simulink model "afe_rst_inv_psm_distributed_control_two_delays"  (R2026a)
settings: Solver=ode1be  StopTime=simlength  FixedStep=tc  MaxStep=Tc
values from neighbouring files (symbols this model uses):
  Amplitude_U = 1.16    [grid_fault_generator.m]
  Amplitude_V = Amplitude_U    (= 1.16)    [grid_fault_generator.m]
  Amplitude_W = Amplitude_U    (= 1.16)    [grid_fault_generator.m]
  end_time_LVRT = start_time_LVRT + error_length    [grid_fault_generator.m]
  Igrid_phase_normalization_factor = 270*sqrt(2)    [grid_emulator.m]
  omega_grid_emulator_nom = w_grid    (= 314.159265359)    [grid_emulator.m]
  omega_grid_nom = w_grid    (= 314.159265359)    [grid_emulator.m]
  t_ramp = 20e-3    (= 0.02)    [grid_fault_generator.m]
  ugrid_factor = 1    [grid_emulator.m]
  V_phase_normalization_factor = Vgrid_phase_normalization_factor    [grid_emulator.m]
  Vdc_bez = 1070    [grid_emulator.m]
  Vemu_ref_norm = Vemu_ref * sqrt(2) / V_phase_normalization_factor    [grid_emulator.m]
  vn_eta_pu = 0    [grid_emulator.m]
  vn_xi_pu = 0    [grid_emulator.m]
  vp_xi_pu = 1    [grid_emulator.m]
undefined symbols (not defined in the file or in its folder): Adrso, Aresd, Bresd, CFi, CFu, Cresd, Crso, CTRPIFF_CLIP_RELEASE, dead_time_INV, emf_fb_p, emf_fb_p_ccaller_1, emf_fb_p_ccaller_2, emf_p, emf_p_ccaller_1, emf_p_ccaller_2, fPWM_INV, g0_161Hz, g0_500Hz, g1_161Hz, g1_500Hz, i_grid_neg_eta_lim, i_grid_neg_eta_red_lim, i_grid_neg_xi_lim, i_grid_neg_xi_red_lim, i_grid_pos_eta_lim, i_grid_pos_eta_red_lim, ibez, id_lim, ieta_neg_ref_lim, ieta_pos_ref_lim, iq_lim, ixi_pos_ref_lim, Jm_norm, k_frt_ref, kg, ki_afe, ki_i, ki_id, ki_iq, ki_rc_neg_grid, ki_rc_pos_grid, ki_vs, ki_w, kp_afe, kp_i, kp_id, kp_iq, kp_rc_neg_grid, kp_rc_pos_grid, kp_vs, kp_w, kw, l1, l2, Lalpha_norm, Ld_norm, Ldrso, Lq_norm, Ls_norm, luenberger_l1 ... (+30)
libraries: fl_lib x146, nesl_utility x62, simulink x8, cstblocks_lti x7, sl_discontinuities x3, single_phase_transformer_lib x3, flexshaft_lib x1, permanent_magnet_synchronous_machine x1
(part 5 of 14)

== system afe_rst_inv_psm_distributed_control_two_delays/mainboard_afe/sequences_current_control/negative_sequence_xi_current_control ==
  ff : Inport
  e : Inport  Port=2
  1/Ti : Gain  Gain=kp_rc_neg_grid  SaturateOnIntegerOverflow=on  OutDataTypeStr=Inherit: Same as input  ParamDataTypeStr=Inherit: Same as input
  1/Ti1 : Gain  SaturateOnIntegerOverflow=on  OutDataTypeStr=Inherit: Same as input  ParamDataTypeStr=Inherit: Same as input
  Saturation : Saturate  UpperLimit=ieta_pos_ref_lim  LowerLimit=-ieta_pos_ref_lim
  Sum : Sum  Inputs=|++
  Sum2 : Sum  Inputs=+++  SaturateOnIntegerOverflow=on
  Sum3 : Sum  Inputs=-+  SaturateOnIntegerOverflow=on
  Unit Delay1 : UnitDelay  SampleTime=ts_afe
  Unit Delay4 : UnitDelay  SampleTime=ts_afe
  kp : Gain  Gain=ki_rc_neg_grid*ts_afe  SaturateOnIntegerOverflow=on  OutDataTypeStr=Inherit: Same as input  ParamDataTypeStr=Inherit: Same as input
  u : Outport  VectorParamsAs1DForOutWhenUnconnected=off
  wires:
  Unit Delay4/1 -> Sum2/3
  Sum3/1 -> Unit Delay4/1
  kp/1 -> Sum2/2
  Sum2/1 -> Saturation/1
  1/Ti/1 -> Sum2/1, Sum3/1
  Saturation/1 -> Sum/1, Sum3/2
  Sum/1 -> Unit Delay1/1
  ff/1 -> 1/Ti1/1
  1/Ti1/1 -> Sum/2
  e/1 -> 1/Ti/1, kp/1  "e"
  Unit Delay1/1 -> u/1

== system afe_rst_inv_psm_distributed_control_two_delays/mainboard_afe/sequences_current_control/positive_sequence_eta_current_control ==
  ff : Inport
  e : Inport  Port=2
  1/Ti : Gain  Gain=kp_rc_pos_grid  SaturateOnIntegerOverflow=on  OutDataTypeStr=Inherit: Same as input  ParamDataTypeStr=Inherit: Same as input
  1/Ti1 : Gain  SaturateOnIntegerOverflow=on  OutDataTypeStr=Inherit: Same as input  ParamDataTypeStr=Inherit: Same as input
  Saturation : Saturate  UpperLimit=ieta_pos_ref_lim  LowerLimit=-ieta_pos_ref_lim
  Sum : Sum  Inputs=|++
  Sum2 : Sum  Inputs=+++  SaturateOnIntegerOverflow=on
  Sum3 : Sum  Inputs=-+  SaturateOnIntegerOverflow=on
  Unit Delay1 : UnitDelay  SampleTime=ts_afe
  Unit Delay4 : UnitDelay  SampleTime=ts_afe
  kp : Gain  Gain=ki_rc_pos_grid*ts_afe  SaturateOnIntegerOverflow=on  OutDataTypeStr=Inherit: Same as input  ParamDataTypeStr=Inherit: Same as input
  u : Outport  VectorParamsAs1DForOutWhenUnconnected=off
  wires:
  Unit Delay4/1 -> Sum2/3
  Sum3/1 -> Unit Delay4/1
  kp/1 -> Sum2/2
  Sum2/1 -> Saturation/1
  1/Ti/1 -> Sum2/1, Sum3/1
  Saturation/1 -> Sum/1, Sum3/2
  ff/1 -> 1/Ti1/1
  1/Ti1/1 -> Sum/2
  e/1 -> 1/Ti/1, kp/1  "e"
  Sum/1 -> Unit Delay1/1
  Unit Delay1/1 -> u/1

== system afe_rst_inv_psm_distributed_control_two_delays/mainboard_afe/voltage-current-acquisition/iga_fieldbus ==
  is : Inport
  Unit Delay : UnitDelay  SampleTime=ts_afe
  Unit Delay1 : UnitDelay  SampleTime=ts_afe
  Zero-Order Hold : ZeroOrderHold  SampleTime=ts_afe
  is_fb : Outport
  wires:
  is/1 -> Zero-Order Hold/1
  Unit Delay/1 -> Unit Delay1/1
  Zero-Order Hold/1 -> Unit Delay/1
  Unit Delay1/1 -> is_fb/1

== system afe_rst_inv_psm_distributed_control_two_delays/mainboard_afe/voltage-current-acquisition/igb_fieldbus ==
  is : Inport
  Unit Delay : UnitDelay  SampleTime=ts_afe
  Unit Delay1 : UnitDelay  SampleTime=ts_afe
  Zero-Order Hold : ZeroOrderHold  SampleTime=ts_afe
  is_fb : Outport
  wires:
  is/1 -> Zero-Order Hold/1
  Unit Delay/1 -> Unit Delay1/1
  Zero-Order Hold/1 -> Unit Delay/1
  Unit Delay1/1 -> is_fb/1

== system afe_rst_inv_psm_distributed_control_two_delays/mainboard_afe/voltage-current-acquisition/igc_fieldbus ==
  is : Inport
  Unit Delay : UnitDelay  SampleTime=ts_afe
  Unit Delay1 : UnitDelay  SampleTime=ts_afe
  Zero-Order Hold : ZeroOrderHold  SampleTime=ts_afe
  is_fb : Outport
  wires:
  is/1 -> Zero-Order Hold/1
  Unit Delay/1 -> Unit Delay1/1
  Zero-Order Hold/1 -> Unit Delay/1
  Unit Delay1/1 -> is_fb/1

== system afe_rst_inv_psm_distributed_control_two_delays/mainboard_afe/voltage-current-acquisition/isa_fieldbus ==
  is : Inport
  Unit Delay : UnitDelay  SampleTime=ts_afe
  Unit Delay1 : UnitDelay  SampleTime=ts_afe
  Zero-Order Hold : ZeroOrderHold  SampleTime=ts_afe
  is_fb : Outport
  wires:
  is/1 -> Zero-Order Hold/1
  Unit Delay/1 -> Unit Delay1/1
  Zero-Order Hold/1 -> Unit Delay/1
  Unit Delay1/1 -> is_fb/1

== system afe_rst_inv_psm_distributed_control_two_delays/mainboard_afe/voltage-current-acquisition/isb_fieldbus ==
  is : Inport
  Unit Delay : UnitDelay  SampleTime=ts_afe
  Unit Delay1 : UnitDelay  SampleTime=ts_afe
  Zero-Order Hold : ZeroOrderHold  SampleTime=ts_afe
  is_fb : Outport
  wires:
  is/1 -> Zero-Order Hold/1
  Unit Delay/1 -> Unit Delay1/1
  Zero-Order Hold/1 -> Unit Delay/1
  Unit Delay1/1 -> is_fb/1

== system afe_rst_inv_psm_distributed_control_two_delays/mainboard_afe/voltage-current-acquisition/isc_fieldbus ==
  is : Inport
  Unit Delay : UnitDelay  SampleTime=ts_afe
  Unit Delay1 : UnitDelay  SampleTime=ts_afe
  Zero-Order Hold : ZeroOrderHold  SampleTime=ts_afe
  is_fb : Outport
  wires:
  is/1 -> Zero-Order Hold/1
  Unit Delay/1 -> Unit Delay1/1
  Zero-Order Hold/1 -> Unit Delay/1
  Unit Delay1/1 -> is_fb/1

== system afe_rst_inv_psm_distributed_control_two_delays/mainboard_afe/voltage-current-acquisition/uga_fieldbus ==
  ug : Inport
  Unit Delay : UnitDelay  SampleTime=ts_afe
  Unit Delay1 : UnitDelay  SampleTime=ts_afe
  Zero-Order Hold : ZeroOrderHold  SampleTime=ts_afe
  ug_fb : Outport
  wires:
  ug/1 -> Zero-Order Hold/1
  Unit Delay/1 -> Unit Delay1/1
  Zero-Order Hold/1 -> Unit Delay/1
  Unit Delay1/1 -> ug_fb/1

== system afe_rst_inv_psm_distributed_control_two_delays/mainboard_afe/voltage-current-acquisition/ugb_fieldbus ==
  ug : Inport
  Unit Delay : UnitDelay  SampleTime=ts_afe
  Unit Delay1 : UnitDelay  SampleTime=ts_afe
  Zero-Order Hold : ZeroOrderHold  SampleTime=ts_afe
  ug_fb : Outport
  wires:
  ug/1 -> Zero-Order Hold/1
  Unit Delay/1 -> Unit Delay1/1
  Zero-Order Hold/1 -> Unit Delay/1
  Unit Delay1/1 -> ug_fb/1

== system afe_rst_inv_psm_distributed_control_two_delays/mainboard_afe/voltage-current-acquisition/ugb_fieldbus1 ==
  ug : Inport
  Unit Delay : UnitDelay  SampleTime=ts_afe
  Unit Delay1 : UnitDelay  SampleTime=ts_afe
  Zero-Order Hold : ZeroOrderHold  SampleTime=ts_afe
  ug_fb : Outport
  wires:
  ug/1 -> Zero-Order Hold/1
  Unit Delay/1 -> Unit Delay1/1
  Zero-Order Hold/1 -> Unit Delay/1
  Unit Delay1/1 -> ug_fb/1

== system afe_rst_inv_psm_distributed_control_two_delays/mainboard_afe/voltage_sequence_avg/Moving Average Filter1 ==
  In2 : Inport
  In3 : Inport  Port=2
  Bus Selector : BusSelector  OutputSignals=ts,sshort,slong,pinput,cbpointer,cbsample,mavg_output
  C Caller : CCaller  FunctionName=mavgflt_process_simulink  PortSpecificationStruct="%)30     .    B H   8    (     @         %    \"     8    !     0         %  0 \"0    $    _    07)G3F%M90  4&]R=$YA;64 4V-O<&4     26YD97@     5'EP90      4VEZ90      27-';&]B86P   X    P    !@    @    $          4    (     0    ,    !         !   P!O=70 #@   #     &    \"     0         !0    @    !     P    $         $  # &]U=  .    .     8    (    !          %    \"     $    &     0         0   ...(+3251 chars)"  SampleTime=ts_afe
  Compare To Zero : simulink/Logic and Bit Operations/Compare To Zero  relop=>  OutDataTypeStr=boolean
  Constant : Constant
  Constant5 : Constant  Value=ts_afe
  Data Type Conversion : DataTypeConversion  OutDataTypeStr=single  SaturateOnIntegerOverflow=off  RndMeth=Floor
  Data Type Conversion1 : DataTypeConversion  OutDataTypeStr=single  SaturateOnIntegerOverflow=off  RndMeth=Floor
  Data Type Conversion2 : DataTypeConversion  OutDataTypeStr=single  SaturateOnIntegerOverflow=off  RndMeth=Floor
  Data Type Conversion3 : DataTypeConversion  OutDataTypeStr=double  SaturateOnIntegerOverflow=off  RndMeth=Floor
  Data Type Conversion4 : DataTypeConversion  OutDataTypeStr=uint8  SaturateOnIntegerOverflow=off  RndMeth=Floor
  Data Type Conversion5 : DataTypeConversion  OutDataTypeStr=uint8  SaturateOnIntegerOverflow=off  RndMeth=Floor
  Enabled Subsystem : Subsystem  TreatAsAtomicUnit=on
  Reset Trigger : Subsystem
  Terminator{,1..5} (6 alike) : Terminator
  Zero-Order Hold1 : ZeroOrderHold  SampleTime=ts_afe
  Zero-Order Hold2 : ZeroOrderHold  SampleTime=ts_afe
  xi : Outport
  wires:
  Bus Selector/5 -> Terminator2/1  "<cbpointer>"
  Bus Selector/4 -> Terminator1/1  "<pinput>"
  Data Type Conversion3/1 -> xi/1  "output"
  Zero-Order Hold2/1 -> Data Type Conversion/1  "d1"
  Enabled Subsystem/1(Out1) -> Data Type Conversion1/1
  Compare To Zero/1 -> Enabled Subsystem/Enable
  In3/1 -> Enabled Subsystem/1(In1), Compare To Zero/1  "omega_grid"
  Constant5/1 -> Zero-Order Hold1/1
  Zero-Order Hold1/1 -> Data Type Conversion2/1  "d1"
  Bus Selector/3 -> Terminator4/1  "<slong>"
  Bus Selector/2 -> Terminator3/1  "<sshort>"
  Bus Selector/1 -> Terminator/1  "<ts>"
  C Caller/1 -> Bus Selector/1  "out"
  In2/1 -> Zero-Order Hold2/1  "input"
  Data Type Conversion4/1 -> C Caller/5
  Data Type Conversion/1 -> C Caller/1  "input"
  Data Type Conversion5/1 -> C Caller/4
  Data Type Conversion2/1 -> C Caller/3
  Data Type Conversion1/1 -> C Caller/2
  Reset Trigger/1(Out1) -> Data Type Conversion5/1
  Constant/1 -> Data Type Conversion4/1
  Bus Selector/6 -> Terminator5/1  "<cbsample>"
  Bus Selector/7 -> Data Type Conversion3/1  "<mavg_output>"

== system afe_rst_inv_psm_distributed_control_two_delays/mainboard_afe/voltage_sequence_avg/Moving Average Filter2 ==
  In2 : Inport
  In3 : Inport  Port=2
  Bus Selector : BusSelector  OutputSignals=ts,sshort,slong,pinput,cbpointer,cbsample,mavg_output
  C Caller : CCaller  FunctionName=mavgflt_process_simulink  PortSpecificationStruct="%)30     .    B H   8    (     @         %    \"     8    !     0         %  0 \"0    $    _    07)G3F%M90  4&]R=$YA;64 4V-O<&4     26YD97@     5'EP90      4VEZ90      27-';&]B86P   X    P    !@    @    $          4    (     0    ,    !         !   P!O=70 #@   #     &    \"     0         !0    @    !     P    $         $  # &]U=  .    .     8    (    !          %    \"     $    &     0         0   ...(+3251 chars)"  SampleTime=ts_afe
  Compare To Zero : simulink/Logic and Bit Operations/Compare To Zero  relop=>  OutDataTypeStr=boolean
  Constant : Constant  Value=2
  Constant5 : Constant  Value=ts_afe
  Data Type Conversion : DataTypeConversion  OutDataTypeStr=single  SaturateOnIntegerOverflow=off  RndMeth=Floor
  Data Type Conversion1 : DataTypeConversion  OutDataTypeStr=single  SaturateOnIntegerOverflow=off  RndMeth=Floor
  Data Type Conversion2 : DataTypeConversion  OutDataTypeStr=single  SaturateOnIntegerOverflow=off  RndMeth=Floor
  Data Type Conversion3 : DataTypeConversion  OutDataTypeStr=double  SaturateOnIntegerOverflow=off  RndMeth=Floor
  Data Type Conversion4 : DataTypeConversion  OutDataTypeStr=uint8  SaturateOnIntegerOverflow=off  RndMeth=Floor
  Data Type Conversion5 : DataTypeConversion  OutDataTypeStr=uint8  SaturateOnIntegerOverflow=off  RndMeth=Floor
  Enabled Subsystem : Subsystem  TreatAsAtomicUnit=on
  Reset Trigger : Subsystem
  Terminator{,1..5} (6 alike) : Terminator
  Zero-Order Hold1 : ZeroOrderHold  SampleTime=ts_afe
  Zero-Order Hold2 : ZeroOrderHold  SampleTime=ts_afe
  xi : Outport
  wires:
  Bus Selector/7 -> Data Type Conversion3/1  "<mavg_output>"
  Bus Selector/6 -> Terminator5/1  "<cbsample>"
  Constant/1 -> Data Type Conversion4/1
  Reset Trigger/1(Out1) -> Data Type Conversion5/1
  Data Type Conversion1/1 -> C Caller/2
  Data Type Conversion2/1 -> C Caller/3
  Data Type Conversion5/1 -> C Caller/4
  Data Type Conversion/1 -> C Caller/1  "input"
  Data Type Conversion4/1 -> C Caller/5
  In2/1 -> Zero-Order Hold2/1  "input"
  C Caller/1 -> Bus Selector/1  "out"
  Bus Selector/1 -> Terminator/1  "<ts>"
  Bus Selector/2 -> Terminator3/1  "<sshort>"
  Bus Selector/3 -> Terminator4/1  "<slong>"
  Zero-Order Hold1/1 -> Data Type Conversion2/1  "d1"
  Constant5/1 -> Zero-Order Hold1/1
  In3/1 -> Compare To Zero/1, Enabled Subsystem/1(In1)  "omega_grid"
  Compare To Zero/1 -> Enabled Subsystem/Enable
  Enabled Subsystem/1(Out1) -> Data Type Conversion1/1
  Zero-Order Hold2/1 -> Data Type Conversion/1  "d1"
  Data Type Conversion3/1 -> xi/1  "output"
  Bus Selector/4 -> Terminator1/1  "<pinput>"
  Bus Selector/5 -> Terminator2/1  "<cbpointer>"

== system afe_rst_inv_psm_distributed_control_two_delays/mainboard_afe/voltage_sequence_avg/Moving Average Filter3 ==
  In2 : Inport
  In3 : Inport  Port=2
  Bus Selector : BusSelector  OutputSignals=ts,sshort,slong,pinput,cbpointer,cbsample,mavg_output
  C Caller : CCaller  FunctionName=mavgflt_process_simulink  PortSpecificationStruct="%)30     .    B H   8    (     @         %    \"     8    !     0         %  0 \"0    $    _    07)G3F%M90  4&]R=$YA;64 4V-O<&4     26YD97@     5'EP90      4VEZ90      27-';&]B86P   X    P    !@    @    $          4    (     0    ,    !         !   P!O=70 #@   #     &    \"     0         !0    @    !     P    $         $  # &]U=  .    .     8    (    !          %    \"     $    &     0         0   ...(+3251 chars)"  SampleTime=ts_afe
  Compare To Zero : simulink/Logic and Bit Operations/Compare To Zero  relop=>  OutDataTypeStr=boolean
  Constant : Constant  Value=3
  Constant5 : Constant  Value=ts_afe
  Data Type Conversion : DataTypeConversion  OutDataTypeStr=single  SaturateOnIntegerOverflow=off  RndMeth=Floor
  Data Type Conversion1 : DataTypeConversion  OutDataTypeStr=single  SaturateOnIntegerOverflow=off  RndMeth=Floor
  Data Type Conversion2 : DataTypeConversion  OutDataTypeStr=single  SaturateOnIntegerOverflow=off  RndMeth=Floor
  Data Type Conversion3 : DataTypeConversion  OutDataTypeStr=double  SaturateOnIntegerOverflow=off  RndMeth=Floor
  Data Type Conversion4 : DataTypeConversion  OutDataTypeStr=uint8  SaturateOnIntegerOverflow=off  RndMeth=Floor
  Data Type Conversion5 : DataTypeConversion  OutDataTypeStr=uint8  SaturateOnIntegerOverflow=off  RndMeth=Floor
  Enabled Subsystem : Subsystem  TreatAsAtomicUnit=on
  Reset Trigger : Subsystem
  Terminator{,1..5} (6 alike) : Terminator
  Zero-Order Hold1 : ZeroOrderHold  SampleTime=ts_afe
  Zero-Order Hold2 : ZeroOrderHold  SampleTime=ts_afe
  xi : Outport
  wires:
  Bus Selector/5 -> Terminator2/1  "<cbpointer>"
  Bus Selector/4 -> Terminator1/1  "<pinput>"
  Data Type Conversion3/1 -> xi/1  "output"
  Zero-Order Hold2/1 -> Data Type Conversion/1  "d1"
  Enabled Subsystem/1(Out1) -> Data Type Conversion1/1
  Compare To Zero/1 -> Enabled Subsystem/Enable
  In3/1 -> Enabled Subsystem/1(In1), Compare To Zero/1  "omega_grid"
  Constant5/1 -> Zero-Order Hold1/1
  Zero-Order Hold1/1 -> Data Type Conversion2/1  "d1"
  Bus Selector/3 -> Terminator4/1  "<slong>"
  Bus Selector/2 -> Terminator3/1  "<sshort>"
  Bus Selector/1 -> Terminator/1  "<ts>"
  C Caller/1 -> Bus Selector/1  "out"
  In2/1 -> Zero-Order Hold2/1  "input"
  Data Type Conversion4/1 -> C Caller/5
  Data Type Conversion/1 -> C Caller/1  "input"
  Data Type Conversion5/1 -> C Caller/4
  Data Type Conversion2/1 -> C Caller/3
  Data Type Conversion1/1 -> C Caller/2
  Reset Trigger/1(Out1) -> Data Type Conversion5/1
  Constant/1 -> Data Type Conversion4/1
  Bus Selector/6 -> Terminator5/1  "<cbsample>"
  Bus Selector/7 -> Data Type Conversion3/1  "<mavg_output>"

== system afe_rst_inv_psm_distributed_control_two_delays/mainboard_afe/voltage_sequence_avg/Moving Average Filter4 ==
  In2 : Inport
  In3 : Inport  Port=2
  Bus Selector : BusSelector  OutputSignals=ts,sshort,slong,pinput,cbpointer,cbsample,mavg_output
  C Caller : CCaller  FunctionName=mavgflt_process_simulink  PortSpecificationStruct="%)30     .    B H   8    (     @         %    \"     8    !     0         %  0 \"0    $    _    07)G3F%M90  4&]R=$YA;64 4V-O<&4     26YD97@     5'EP90      4VEZ90      27-';&]B86P   X    P    !@    @    $          4    (     0    ,    !         !   P!O=70 #@   #     &    \"     0         !0    @    !     P    $         $  # &]U=  .    .     8    (    !          %    \"     $    &     0         0   ...(+3251 chars)"  SampleTime=ts_afe
  Compare To Zero : simulink/Logic and Bit Operations/Compare To Zero  relop=>  OutDataTypeStr=boolean
  Constant : Constant  Value=4
  Constant5 : Constant  Value=ts_afe
  Data Type Conversion : DataTypeConversion  OutDataTypeStr=single  SaturateOnIntegerOverflow=off  RndMeth=Floor
  Data Type Conversion1 : DataTypeConversion  OutDataTypeStr=single  SaturateOnIntegerOverflow=off  RndMeth=Floor
  Data Type Conversion2 : DataTypeConversion  OutDataTypeStr=single  SaturateOnIntegerOverflow=off  RndMeth=Floor
  Data Type Conversion3 : DataTypeConversion  OutDataTypeStr=double  SaturateOnIntegerOverflow=off  RndMeth=Floor
  Data Type Conversion4 : DataTypeConversion  OutDataTypeStr=uint8  SaturateOnIntegerOverflow=off  RndMeth=Floor
  Data Type Conversion5 : DataTypeConversion  OutDataTypeStr=uint8  SaturateOnIntegerOverflow=off  RndMeth=Floor
  Enabled Subsystem : Subsystem  TreatAsAtomicUnit=on
  Reset Trigger : Subsystem
  Terminator{,1..5} (6 alike) : Terminator
  Zero-Order Hold1 : ZeroOrderHold  SampleTime=ts_afe
  Zero-Order Hold2 : ZeroOrderHold  SampleTime=ts_afe
  xi : Outport
  wires:
  Bus Selector/7 -> Data Type Conversion3/1  "<mavg_output>"
  Bus Selector/6 -> Terminator5/1  "<cbsample>"
  Constant/1 -> Data Type Conversion4/1
  Reset Trigger/1(Out1) -> Data Type Conversion5/1
  Data Type Conversion1/1 -> C Caller/2
  Data Type Conversion2/1 -> C Caller/3
  Data Type Conversion5/1 -> C Caller/4
  Data Type Conversion/1 -> C Caller/1  "input"
  Data Type Conversion4/1 -> C Caller/5
  In2/1 -> Zero-Order Hold2/1  "input"
  C Caller/1 -> Bus Selector/1  "out"
  Bus Selector/1 -> Terminator/1  "<ts>"
  Bus Selector/2 -> Terminator3/1  "<sshort>"
  Bus Selector/3 -> Terminator4/1  "<slong>"
  Zero-Order Hold1/1 -> Data Type Conversion2/1  "d1"
  Constant5/1 -> Zero-Order Hold1/1
  In3/1 -> Compare To Zero/1, Enabled Subsystem/1(In1)  "omega_grid"
  Compare To Zero/1 -> Enabled Subsystem/Enable
  Enabled Subsystem/1(Out1) -> Data Type Conversion1/1
  Zero-Order Hold2/1 -> Data Type Conversion/1  "d1"
  Data Type Conversion3/1 -> xi/1  "output"
  Bus Selector/4 -> Terminator1/1  "<pinput>"
  Bus Selector/5 -> Terminator2/1  "<cbpointer>"

== system afe_rst_inv_psm_distributed_control_two_delays/AFE-Modular/afe_leg_a/driver_board_a/current_ctrl ==
  i_xi_ref : Inport
  phase_current_control : Subsystem
  xieta2abc : Subsystem
  us_alphabeta_ctrl : Outport
  wires:
  i_xi_ref/1 -> xieta2abc/1(pos_xi)  "i_xi_ref"
  phase_current_control/1(us_alphabeta_ctrl) -> us_alphabeta_ctrl/1
  xieta2abc/1(i_abc) -> phase_current_control/1(In1)  "is_abc_reference"
  [gamma_grid_phase_a] -> xieta2abc/5(gamma)
  [isa_pu_dba] -> phase_current_control/2(is_abc)
  [is_eta_pos_ref_mb_fb_dba] -> xieta2abc/2(pos_eta)
  [is_xi_neg_ref_mb_fb_dba] -> xieta2abc/3(neg_xi)
  [is_eta_neg_ref_mb_fb_dba] -> xieta2abc/4(neg_eta)

== system afe_rst_inv_psm_distributed_control_two_delays/AFE-Modular/afe_leg_a/driver_board_a/dq_pll ==
  pll_stageA : Subsystem
  pll_stageB : Subsystem
  tag scope: gamma_grid_phase_a=global
  wires:
  pll_stageB/1(gamma_grid_pll) -> pll_stageA/1(gamma_grid), [gamma_grid_phase_a]
  pll_stageA/2(u_grid_pos_eta) -> pll_stageB/2(u_grid_pos_eta)  "u_grid_pos_eta"
  pll_stageA/1(u_grid_pos_xi) -> pll_stageB/1(u_grid_pos_xi)  "u_grid_pos_xi"

== system afe_rst_inv_psm_distributed_control_two_delays/AFE-Modular/afe_leg_a/driver_board_a/iga_dba_estimator ==
  Gain : Gain  Gain=omega_grid_nom*CFu
  Sum : Sum  Inputs=|++
  quadrature_shift_filter : MATLAB Function  TreatAsAtomicUnit=on  SystemSampleTime=ts_afe
  tag scope: iga_pu_dba=global
  wires:
  Sum/1 -> [iga_pu_dba]
  quadrature_shift_filter/1(y) -> Sum/2
  [uga_pu_dba] -> Gain/1
  [isa_pu_dba] -> Sum/1
  Gain/1 -> quadrature_shift_filter/1(input)

== system afe_rst_inv_psm_distributed_control_two_delays/AFE-Modular/afe_leg_a/driver_board_a/udc_ctrl ==
  udc_pu : Inport
  udc_pu_ref : Inport  Port=2
  1/Ti : Gain  Gain=kp_vs  SaturateOnIntegerOverflow=on  OutDataTypeStr=Inherit: Same as input  ParamDataTypeStr=Inherit: Same as input
  Gain : Gain  Gain=-1
  Saturation : Saturate  UpperLimit=ixi_pos_ref_lim  LowerLimit=-ixi_pos_ref_lim
  Sum1 : Sum  Inputs=+++  SaturateOnIntegerOverflow=on
  Sum2 : Sum  Inputs=-+  SaturateOnIntegerOverflow=on
  Sum3 : Sum  Inputs=-+  SaturateOnIntegerOverflow=on
  Unit Delay4 : UnitDelay  SampleTime=ts_afe
  kp : Gain  Gain=ki_vs*ts_afe  SaturateOnIntegerOverflow=on  OutDataTypeStr=Inherit: Same as input  ParamDataTypeStr=Inherit: Same as input
  i_xi_ref : Outport
  wires:
  1/Ti/1 -> Sum1/1, Sum3/1
  kp/1 -> Sum1/2
  Sum3/1 -> Unit Delay4/1
  Unit Delay4/1 -> Sum1/3
  udc_pu_ref/1 -> Sum2/2
  udc_pu/1 -> Sum2/1
  Sum2/1 -> kp/1, 1/Ti/1
  Sum1/1 -> Saturation/1
  Saturation/1 -> Gain/1, Sum3/2
  Gain/1 -> i_xi_ref/1

== system afe_rst_inv_psm_distributed_control_two_delays/AFE-Modular/afe_leg_a/driver_board_a/voltage-current-acquisition ==
  is_eta_neg_ref_fieldbus : Subsystem
  is_eta_pos_ref_fieldbus : Subsystem
  is_xi_neg_ref_fieldbus : Subsystem
  isa_measure : Subsystem
  isb_fieldbus : Subsystem
  isc_fieldbus : Subsystem
  ixi_ref_fieldbus : Subsystem
  ixi_ref_fieldbus1 : Subsystem
  ub_ctrl_fieldbus : Subsystem
  uc_ctrl_fieldbus : Subsystem
  uga_measure : Subsystem
  ugb_fieldbus : Subsystem
  ugc_fieldbus : Subsystem
  tag scope: is_eta_neg_ref_mb_fb_dba=global, is_eta_pos_ref_mb_fb_dba=global, is_xi_neg_ref_mb_fb_dba=global, isa_pu_dba=global, isb_pu_dbb_fb_dba=global, isc_pu_dbc_fb_dba=global, ixi_ref_dbb_fb_dba=global, ixi_ref_dbc_fb_dba=global, uga_pu_dba=global, ugb_pu_dbb_fb_dba=global, ugc_pu_dbc_fb_dba=global, usb_ctrl_dbb_fb_dba=global, usc_ctrl_dbc_fb_dba=global
  wires:
  ub_ctrl_fieldbus/1(u_ctrl_fb) -> [usb_ctrl_dbb_fb_dba]
  [isc_pu_dbc] -> isc_fieldbus/1(is)
  isb_fieldbus/1(is_fb) -> [isb_pu_dbb_fb_dba]
  [usc_ctrl_dbc] -> uc_ctrl_fieldbus/1(u_ctrl)
  isa_measure/1(is_pu) -> [isa_pu_dba]
  [isb_pu_dbb] -> isb_fieldbus/1(is)
  [usb_ctrl_dbb] -> ub_ctrl_fieldbus/1(u_ctrl)
  [isa_dba] -> isa_measure/1(is)
  uc_ctrl_fieldbus/1(u_ctrl_fb) -> [usc_ctrl_dbc_fb_dba]
  isc_fieldbus/1(is_fb) -> [isc_pu_dbc_fb_dba]
  [uga_dba] -> uga_measure/1(ug)
  uga_measure/1(ug_pu) -> [uga_pu_dba]
  [ugc_pu_dbc] -> ugc_fieldbus/1(ug)
  [ugb_pu_dbb] -> ugb_fieldbus/1(ug)
  ugc_fieldbus/1(ug_fb) -> [ugc_pu_dbc_fb_dba]
  ugb_fieldbus/1(ug_fb) -> [ugb_pu_dbb_fb_dba]
  ixi_ref_fieldbus/1(is_fb) -> [ixi_ref_dbb_fb_dba]
  ixi_ref_fieldbus1/1(is_fb) -> [ixi_ref_dbc_fb_dba]
  [ixi_ref_dbc] -> ixi_ref_fieldbus1/1(is)
  [ixi_ref_dbb] -> ixi_ref_fieldbus/1(is)
  [i_stack_pos_eta_ref] -> is_eta_pos_ref_fieldbus/1(is)
  is_eta_pos_ref_fieldbus/1(is_fb) -> [is_eta_pos_ref_mb_fb_dba]
  [i_stack_neg_eta_ref] -> is_eta_neg_ref_fieldbus/1(is)
  is_eta_neg_ref_fieldbus/1(is_fb) -> [is_eta_neg_ref_mb_fb_dba]
  [i_stack_neg_xi_ref] -> is_xi_neg_ref_fieldbus/1(is)
  is_xi_neg_ref_fieldbus/1(is_fb) -> [is_xi_neg_ref_mb_fb_dba]

== system afe_rst_inv_psm_distributed_control_two_delays/AFE-Modular/afe_leg_a/modulator/sv_pwm ==
  ab : Inport
  enable : Inport  Port=2
  Bus Selector : BusSelector  OutputSignals=da,db,dc
  Bus Selector1 : BusSelector  OutputSignals=us_alpha_ctrl,us_beta_ctrl
  C Caller : CCaller  FunctionName=sv_pwm_process_simulink  PortSpecificationStruct="%)30     .    N @   8    (     @         %    \"     4    !     0         %  0 \"0    $    _    07)G3F%M90  4&]R=$YA;64 4V-O<&4     26YD97@     5'EP90      4VEZ90      27-';&]B86P   X    P    !@    @    $          4    (     0    ,    !         !   P!O=70 #@   #     &    \"     0         !0    @    !     P    $         $  # &]U=  .    .     8    (    !          %    \"     $    &     0         0   ...(+2630 chars)"  SampleTime=ts_afe
  Constant : Constant  Value=ts_afe
  Data Type Conversion1 : DataTypeConversion  OutDataTypeStr=double  SaturateOnIntegerOverflow=off  RndMeth=Floor
  Data Type Conversion15 : DataTypeConversion  OutDataTypeStr=single  SaturateOnIntegerOverflow=off  RndMeth=Floor
  Data Type Conversion16 : DataTypeConversion  OutDataTypeStr=single  SaturateOnIntegerOverflow=off  RndMeth=Floor
  Data Type Conversion17 : DataTypeConversion  OutDataTypeStr=uint32  SaturateOnIntegerOverflow=off  RndMeth=Floor
  Data Type Conversion18 : DataTypeConversion  OutDataTypeStr=single  SaturateOnIntegerOverflow=off  RndMeth=Floor
  Data Type Conversion2 : DataTypeConversion  OutDataTypeStr=double  SaturateOnIntegerOverflow=off  RndMeth=Floor
  Data Type Conversion3 : DataTypeConversion  OutDataTypeStr=double  SaturateOnIntegerOverflow=off  RndMeth=Floor
  Zero-Order Hold{,1..3} (4 alike) : ZeroOrderHold  SampleTime=ts_afe
  alphabeta2uvw : MATLAB Function  TreatAsAtomicUnit=on  SystemSampleTime=ts_afe
  modulator : Subsystem
  firing_gates : Outport
  tag scope: afe_mu=global, afe_mv=global, afe_mw=global
  wires:
  Zero-Order Hold/1 -> C Caller/1
  Zero-Order Hold2/1 -> C Caller/3
  Constant/1 -> Data Type Conversion16/1
  Data Type Conversion18/1 -> Zero-Order Hold/1
  enable/1 -> Data Type Conversion17/1
  Data Type Conversion16/1 -> Zero-Order Hold2/1
  Zero-Order Hold1/1 -> C Caller/2
  Data Type Conversion17/1 -> Zero-Order Hold3/1
  Zero-Order Hold3/1 -> C Caller/4
  Data Type Conversion15/1 -> Zero-Order Hold1/1
  C Caller/1 -> Bus Selector/1  "out"
  modulator/1(firing_gates) -> firing_gates/1
  ab/1 -> Bus Selector1/1
  Bus Selector1/1 -> alphabeta2uvw/1(alpha), Data Type Conversion18/1  "<us_alpha_ctrl>"
  Bus Selector1/2 -> alphabeta2uvw/2(beta), Data Type Conversion15/1  "<us_beta_ctrl>"
  Data Type Conversion3/1 -> modulator/3(w)  "dw"
  Data Type Conversion2/1 -> modulator/2(v)  "dv"
  Data Type Conversion1/1 -> modulator/1(u)  "du"
  Bus Selector/1 -> Data Type Conversion1/1  "<da>"
  Bus Selector/2 -> Data Type Conversion2/1  "<db>"
  Bus Selector/3 -> Data Type Conversion3/1  "<dc>"
  alphabeta2uvw/2(v) -> [afe_mv]  "mv"
  alphabeta2uvw/1(u) -> [afe_mu]  "mu"
  alphabeta2uvw/3(w) -> [afe_mw]  "mw"

== system afe_rst_inv_psm_distributed_control_two_delays/AFE-Modular/afe_leg_a/solid_state_inverter/switch_1 ==
  Diode : fl_lib/Electrical/Electrical Elements/Diode  Vf=Vgamma V  Ron=Ron Ohm  Goff=1e-8 1/Ohm  i_specify=off  i_priority=None  i=0 A  i_nominal_specify=off  i_nominal_value=1  i_nominal_unit=A  v_specify=off  v_priority=None  v=0 V  v_nominal_specify=off  v_nominal_value=1  v_nominal_unit=V
  Switch : fl_lib/Electrical/Electrical Elements/Switch  R_closed=Ron Ohm  G_open=1e-8 1/Ohm  Threshold=7.5  i_specify=off  i_priority=None  i=0 A  i_nominal_specify=off  i_nominal_value=1  i_nominal_unit=A  v_specify=off  v_priority=None  v=0 V  v_nominal_specify=off  v_nominal_value=1  v_nominal_unit=V
  snubber : fl_lib/Electrical/Electrical Elements/Capacitor  c=Csnubber F  r=Rsnubber Ohm  g=0 1/Ohm  i_specify=off  i_priority=None  i=0 A  i_nominal_specify=off  i_nominal_value=1  i_nominal_unit=A  v_specify=off  v_priority=None  v=0 V  v_nominal_specify=off  v_nominal_value=1  v_nominal_unit=V  vc_specify=off  vc_priority=High  vc=0 V  vc_nominal_specify=off  vc_nominal_value=1  vc_nominal_unit=V
  G : PMIOPort  Side=Left
  C : PMIOPort  Port=2  Side=Left
  E : PMIOPort  Port=3  Side=Right
  connections:
  Switch/RConn2 -- C/RConn1 -- snubber/LConn1 -- Diode/RConn1
  Switch/RConn1 -- G/RConn1
  Switch/LConn1 -- E/RConn1 -- snubber/RConn1 -- Diode/LConn1

== system afe_rst_inv_psm_distributed_control_two_delays/AFE-Modular/afe_leg_a/solid_state_inverter/switch_2 ==
  Diode : fl_lib/Electrical/Electrical Elements/Diode  Vf=Vgamma V  Ron=Ron Ohm  Goff=1e-8 1/Ohm  i_specify=off  i_priority=None  i=0 A  i_nominal_specify=off  i_nominal_value=1  i_nominal_unit=A  v_specify=off  v_priority=None  v=0 V  v_nominal_specify=off  v_nominal_value=1  v_nominal_unit=V
  Switch : fl_lib/Electrical/Electrical Elements/Switch  R_closed=Ron Ohm  G_open=1e-8 1/Ohm  Threshold=7.5  i_specify=off  i_priority=None  i=0 A  i_nominal_specify=off  i_nominal_value=1  i_nominal_unit=A  v_specify=off  v_priority=None  v=0 V  v_nominal_specify=off  v_nominal_value=1  v_nominal_unit=V
  snubber : fl_lib/Electrical/Electrical Elements/Capacitor  c=Csnubber F  r=Rsnubber Ohm  g=0 1/Ohm  i_specify=off  i_priority=None  i=0 A  i_nominal_specify=off  i_nominal_value=1  i_nominal_unit=A  v_specify=off  v_priority=None  v=0 V  v_nominal_specify=off  v_nominal_value=1  v_nominal_unit=V  vc_specify=off  vc_priority=High  vc=0 V  vc_nominal_specify=off  vc_nominal_value=1  vc_nominal_unit=V
  G : PMIOPort  Side=Left
  C : PMIOPort  Port=2  Side=Left
  E : PMIOPort  Port=3  Side=Right
  connections:
  E/RConn1 -- Switch/LConn1 -- snubber/RConn1 -- Diode/LConn1
  Switch/RConn1 -- G/RConn1
  C/RConn1 -- Switch/RConn2 -- snubber/LConn1 -- Diode/RConn1

== system afe_rst_inv_psm_distributed_control_two_delays/AFE-Modular/afe_leg_b/driver_board_b/current_ctrl ==
  i_xi_ref : Inport
  phase_current_control : Subsystem
  xieta2abc : Subsystem
  us_alphabeta_ctrl : Outport
  wires:
  i_xi_ref/1 -> xieta2abc/1(pos_xi)  "i_xi_ref"
  phase_current_control/1(us_alphabeta_ctrl) -> us_alphabeta_ctrl/1
  xieta2abc/1(i_abc_reference) -> phase_current_control/1(In1)
  [gamma_grid_dbb] -> xieta2abc/5(gamma)
  [isb_pu_dbb] -> phase_current_control/2(is_abc)
  [is_eta_pos_ref_mb_fb_dbb] -> xieta2abc/2(pos_eta)
  [is_xi_neg_ref_mb_fb_dbb] -> xieta2abc/3(neg_xi)
  [is_eta_neg_ref_mb_fb_dbb] -> xieta2abc/4(neg_eta)

== system afe_rst_inv_psm_distributed_control_two_delays/AFE-Modular/afe_leg_b/driver_board_b/dq_pll ==
  pll_stageA : Subsystem
  pll_stageB : Subsystem
  tag scope: gamma_grid_dbb=global
  wires:
  pll_stageB/1(gamma_grid_pll) -> pll_stageA/1(gamma_grid), [gamma_grid_dbb]
  pll_stageA/2(u_grid_pos_eta) -> pll_stageB/2(u_grid_pos_eta)  "u_grid_pos_eta"
  pll_stageA/1(u_grid_pos_xi) -> pll_stageB/1(u_grid_pos_xi)  "u_grid_pos_xi"

== system afe_rst_inv_psm_distributed_control_two_delays/AFE-Modular/afe_leg_b/driver_board_b/igb_dbb_estimator ==
  Gain : Gain  Gain=omega_grid_nom*CFu
  Sum : Sum  Inputs=|++
  quadrature_shift_filter : MATLAB Function  TreatAsAtomicUnit=on  SystemSampleTime=ts_afe
  tag scope: igb_pu_dbb=global
  wires:
  Sum/1 -> [igb_pu_dbb]
  quadrature_shift_filter/1(y) -> Sum/2
  [ugb_pu_dbb] -> Gain/1
  [isb_pu_dbb] -> Sum/1
  Gain/1 -> quadrature_shift_filter/1(input)

== system afe_rst_inv_psm_distributed_control_two_delays/AFE-Modular/afe_leg_b/driver_board_b/voltage-current-acquisition ==
  is_eta_neg_ref_fieldbus : Subsystem
  is_eta_pos_ref_fieldbus : Subsystem
  is_xi_neg_ref_fieldbus : Subsystem
  isa_measure : Subsystem
  isb_fieldbus : Subsystem
  isc_fieldbus : Subsystem
  ixi_ref_fieldbus : Subsystem
  ixi_ref_fieldbus1 : Subsystem
  ub_ctrl_fieldbus : Subsystem
  uc_ctrl_fieldbus : Subsystem
  uga_measure : Subsystem
  ugb_fieldbus : Subsystem
  ugc_fieldbus : Subsystem
  tag scope: is_eta_neg_ref_mb_fb_dbb=global, is_eta_pos_ref_mb_fb_dbb=global, is_xi_neg_ref_mb_fb_dbb=global, isa_pu_dba_fb_dbb=global, isb_pu_dbb=global, isc_pu_dbc_fb_dbb=global, ixi_ref_dba_fb_dbb=global, ixi_ref_dbc_fb_dbb=global, uga_pu_dba_fb_dbb=global, ugb_pu_dbb=global, ugc_pu_dbc_fb_dbb=global, usa_ctrl_dba_fb_dbb=global, usc_ctrl_dbc_fb_dbb=global
  wires:
  ub_ctrl_fieldbus/1(u_ctrl_fb) -> [usa_ctrl_dba_fb_dbb]
  [isc_pu_dbc] -> isc_fieldbus/1(is)
  isb_fieldbus/1(is_fb) -> [isa_pu_dba_fb_dbb]
  [usc_ctrl_dbc] -> uc_ctrl_fieldbus/1(u_ctrl)
  isa_measure/1(is_pu) -> [isb_pu_dbb]
  [isa_pu_dba] -> isb_fieldbus/1(is)
  [usa_ctrl_dba] -> ub_ctrl_fieldbus/1(u_ctrl)
  [isb_dbb] -> isa_measure/1(is)
  uc_ctrl_fieldbus/1(u_ctrl_fb) -> [usc_ctrl_dbc_fb_dbb]
  isc_fieldbus/1(is_fb) -> [isc_pu_dbc_fb_dbb]
  [ugb_dbb] -> uga_measure/1(ug)
  uga_measure/1(ug_pu) -> [ugb_pu_dbb]
  [ugc_pu_dbc] -> ugc_fieldbus/1(ug)
  [uga_pu_dba] -> ugb_fieldbus/1(ug)
  ugc_fieldbus/1(ug_fb) -> [ugc_pu_dbc_fb_dbb]
  ugb_fieldbus/1(ug_fb) -> [uga_pu_dba_fb_dbb]
  [ixi_ref_dba] -> ixi_ref_fieldbus/1(is)
  ixi_ref_fieldbus/1(is_fb) -> [ixi_ref_dba_fb_dbb]
  ixi_ref_fieldbus1/1(is_fb) -> [ixi_ref_dbc_fb_dbb]
  [ixi_ref_dbc] -> ixi_ref_fieldbus1/1(is)
  [i_stack_pos_eta_ref] -> is_eta_pos_ref_fieldbus/1(is)
  [i_stack_neg_eta_ref] -> is_eta_neg_ref_fieldbus/1(is)
  [i_stack_neg_xi_ref] -> is_xi_neg_ref_fieldbus/1(is)
  is_eta_pos_ref_fieldbus/1(is_fb) -> [is_eta_pos_ref_mb_fb_dbb]
  is_eta_neg_ref_fieldbus/1(is_fb) -> [is_eta_neg_ref_mb_fb_dbb]
  is_xi_neg_ref_fieldbus/1(is_fb) -> [is_xi_neg_ref_mb_fb_dbb]
